simulink model "EMT"  (R2024b)
settings: Solver=ode5  StartTime=0.0  StopTime=1500  FixedStep=0.002  RelTol=1e-3
PreLoadFcn:
  | parameter;
InitFcn:
  | parameter;
StopFcn:
  | save('result.mat');
values from neighbouring files (symbols this model uses):
  A = 7.3    [parameter.m]
  a11 = (1+k1)*(1+k2)/k1/k2/iq    (= 1.54241568346)    [parameter.m]
  a11_L = a11    (= 1.54241568346)    [parameter.m]
  a12 = -(1+k1+k2)*(1+k3)/k1/k2    (= -3.86074191629)    [parameter.m]
  a12_L = a11*(1+k3+k4)/(1+k3)    (= 2.43173643789)    [parameter.m]
  a21 = -(1+k2)/k1/iq    (= -1.04963112005)    [parameter.m]
  a22 = (1+k1+k2)/k1    (= 2.46948356808)    [parameter.m]
  B = 2.71    [parameter.m]
  b11 = 0    [parameter.m]
  b12 = (1+k3)    (= 3.33)    [parameter.m]
  b21 = (1+k2)/iq    (= 2.23571428571)    [parameter.m]
  b22 = -k2    (= -2.13)    [parameter.m]
  C1_shift = 200    [parameter.m]
  Cb = 70    [parameter.m]
  Cd = 0.6    [parameter.m]
  eff_generator = eff_motor    [parameter.m]
  eff_motor = [0.80 0.80 0.84 0.84 0.83 0.85 0.83 0.83 0.83 0.80 0.80 0.80 ... (first row only)    [parameter.m]
  ele_map = [10.00,11.46,14.13,19.24,20.94,23.21,20.29,20.23,22.28,17.66,16.24,18.95,20.79,16.98,18.22,16.52,18.29,20.67,20.82,23.14,23.36,21.30,17.71,20.26,19.53,21.18,23.13,22.79,19.35,16.77,20.50,19.02,20.56,21.90,23.91,20.40,18.45,22.70,22.38,22.48,21.84,17.76,20.13,22.61,19.35,19.36,21.56,20.37,18.38,17.96,18.38,17.24,18.99,22.31,23.50,18.24,22.11,20.73,20.35,18.91,22.88,20.92,18.75,16.85,21.94,17.80,19. ...(+2007 chars)    [parameter.m]
  Fb_max = 5.5*mass    (= 247500)    [parameter.m]
  ic = 4.42    [parameter.m]
  JA = 0.4    [parameter.m]
  JB = JA    (= 0.4)    [parameter.m]
  Jc3r4 = 1e-2    (= 0.01)    [parameter.m]
  Je = 2.5    [parameter.m]
  Jh = 1e-2    (= 0.01)    [parameter.m]
  kh = 2.88    [parameter.m]
  kt = 1.83    [parameter.m]
  L = 4.472    [parameter.m]
  mass = 45000    [parameter.m]
  miu_max = 0.8    [parameter.m]
  n_generator = n_motor    [parameter.m]
  n_motor = [0 0.1 0.25 0.4 0.55 0.7 0.85 1 1.15 1.3 1.45 2.2]*3185    [parameter.m]
  nA_map = [-6000:50:-3250 -3200 0 3200 3250:50:6000]    [parameter.m]    (also in plot_result.m = [-7000:50:-3250 -3200 0 3200 3250:50:7000])
  nA_max = max(nA_map)    [parameter.m]
  nA_min = min(nA_map)    [parameter.m]
  nB_map = nA_map    [parameter.m]    (also in plot_result.m = [-7000:50:-3250 -3200 0 3200 3250:50:7000])
  nB_max = nA_max    [parameter.m]
  nB_min = nA_min    [parameter.m]
  ne_idl = 3000    [parameter.m]
  ne_map = [1600,1700,1800,1900,2000,2100,2200,2300,2400,2500,2600,2700,2800,2900,3000,3100,3200,3300,3400,3500,3600,3700,3800,3900,4000,4100,4200,4500]    [parameter.m]
  ne_max = 4200    [parameter.m]
  ne_min = 1600    [parameter.m]
  ne_start = 200    [parameter.m]
  nZ_map = [-8000:50:-4850 -4800 0 4800 4850:50:8000]    [parameter.m]
  Pb_epr = [-45 -45 -40 -30 0 30 40 45 45]    [parameter.m]
  Pb_max = [0 40 45 45 45]    [parameter.m]
  Pb_min = [-45 -45 -45 -40 0]    [parameter.m]
  Pe_ass = 210+20    (= 230)    [parameter.m]
  Pe_max = 1103    [parameter.m]
  PN0 = 0    [parameter.m]
  R_map = [0.90 0.89 0.90 0.91 0.92 0.93 0.94 0.95 0.96 0.97 0.98]/10    [parameter.m]
  rz = 0.318    [parameter.m]
  SOC0 = 60    [parameter.m]
  SOC_epr = [30 31 50 59 60 61 70 79 80]    [parameter.m]
  SOC_map = 0:10:100    [parameter.m]
  T_generator = T_motor    [parameter.m]
  T_motor = [0 0.3 0.8 1.3 1.8 2.3 2.8]/1.8*1110    [parameter.m]
  TA_max_map = [370*9549./(6000:-50:3250) 1110 1110 1110 370*9549./(3250:50:6000)]    [parameter.m]    (also in plot_result.m = [370*9549./(7000:-50:3250) 1100 1100 1100 370*9549./(3250:50)
  TA_min_map = -TA_max_map    [parameter.m]
  TAf = 0    [parameter.m]
  TB_max_map = TA_max_map    [parameter.m]    (also in plot_result.m = [370*9549./(7000:-50:3250) 1110 1110 1110 370*9549./(3250:50)
  TB_min_map = TA_min_map    [parameter.m]
  TBf = TAf    (= 0)    [parameter.m]
  Te_map = [0,599,798,998,1168,1324,1495,1660,1822,1970,2106,2235,2355,2458,2508,2543,2565,2606,2613,2649,2658,2689,2701,2707,2719,2724,2728,2740,2743,2754]    [parameter.m]
  Te_max_map = [1168,1324,1495,1660,1822,1970,2106,2235,2355,2458,2543,2606,2658,2701,2728,2743,2754,2743,2740,2724,2719,2707,2689,2649,2613,2565,2508,998]    [parameter.m]
  Te_start = 1600    [parameter.m]
  Tef = 100    [parameter.m]
  Time = 0:0.1:200    [parameter.m]
  Time_ele = 0:4:1600    [parameter.m]
  TS_A = 0.2    [parameter.m]
  TS_B = TS_A    (= 0.2)    [parameter.m]
  TS_C0 = 0.2    [parameter.m]
  TS_C1 = 0.2    [parameter.m]
  Ts_e = 0.1    [parameter.m]
  TS_Z1 = 0.2    [parameter.m]
  TS_Z2 = 0.2    [parameter.m]
  TZ_max_map = [450*9549./(8000:-50:4850) 1000 1000 1000 450*9549./(4850:50:8000)]    [parameter.m]
  TZ_min_map = -TZ_max_map    [parameter.m]
  Uoc_map = [3.258,3.668,3.733,3.783,3.833,3.877,3.912,3.941,3.973,4.013,4.200]*250    [parameter.m]
  v_cyc = 0.*(0<=Time&Time<11)+(3.75.*Time-41.25).*(11<=Time&Time<15)+15.*(15<=Time&Time<23)+(-3.*Time+84).*(23<=Time&Time<28)+0.*(28<=Time&Time<49)+(8.*Time/3-392/3).*(49<=Time&Time<61)+32.*(61<=Time&Time<85)+(-32.*Time/11+3072/11).*(85<=Time&Time<96)+0.*(96<=Time&Time<117)+(25.*Time/13-2925/13).*(117<=Time&Time<143)+50.*(143<=Time&Time<155)+(-15.*Time/8+2725/8).*(155<=Time&Time<163)+35.*(163<=Time&Time<17 ...(+70 chars)    [parameter.m]
  V_Shift12 = 32    [parameter.m]
  V_Shift21 = 25    [parameter.m]
  Voltage_epr = [750 760 900 1000 1050]    [parameter.m]
  Y_engine = 0.955    [parameter.m]
  Yc = 0.98    [parameter.m]
  Yh = 0.96    [parameter.m]
  Z1_shift = 200    [parameter.m]
  Z2_shift = 200    [parameter.m]
undefined symbols (not defined in the file or in its folder): sigbuilder_block
libraries: fl_lib x82, nesl_utility x55, simulink x49, sdl_lib x10, simulink_need_slupdate x6, powerlib_extras x1
(part 3 of 6)

== system EMT/Control Unit/Control/Power Distribution/Feasible Control Range ==
  stage : Inport
  ne_act : Inport  Port=2
  v_act : Inport  Port=3
  Memory1 : Memory
  Memory5 : Memory
  State Calculation : Subsystem
  State Predition : Subsystem
  stage_k : Outport
  ne_k : Outport  Port=2
  no_k : Outport  Port=3
  Te_k : Outport  Port=4
  TA_k : Outport  Port=5
  TB_k : Outport  Port=6
  wires:
  State Predition/3(no_k) -> no_k/1
  State Predition/4(Te_k) -> Te_k/1
  State Predition/5(TA_k) -> TA_k/1
  State Predition/6(TB_k) -> TB_k/1
  State Predition/2(ne_k) -> ne_k/1
  State Predition/1(stage_k) -> stage_k/1
  ne_act/1 -> Memory5/1
  stage/1 -> State Calculation/1(s)
  v_act/1 -> Memory1/1
  Memory5/1 -> State Calculation/2(ne)
  Memory1/1 -> State Calculation/3(v_act)
  State Calculation/1(stage) -> State Predition/1(stage)
  State Calculation/2(ne_act) -> State Predition/2(ne_act)
  State Calculation/3(nA_act) -> State Predition/3(nA_act)
  State Calculation/4(nB_act) -> State Predition/4(nB_act)
  State Calculation/5(no_act) -> State Predition/5(no_act)

== system EMT/Control Unit/Control/Power Distribution/Oil Control ==
  Demux : Demux
      settings: DisplayOption=none
  Transfer Fcn1 : TransferFcn  Denominator=[TS_C0 1]
  Transfer Fcn2 : TransferFcn  Denominator=[TS_Z1 1]
  Transfer Fcn3 : TransferFcn  Denominator=[TS_Z2 1]
  Transfer Fcn4 : TransferFcn  Denominator=[TS_C1 1]
  tag scope: Press_C0=global, Press_C1=global, Press_Z1=global, Press_Z2=global
  wires:
  Transfer Fcn1/1 -> [Press_C0]
  Transfer Fcn2/1 -> [Press_Z1]
  Demux/1 -> Transfer Fcn1/1
  Demux/4 -> Transfer Fcn4/1
  Demux/3 -> Transfer Fcn3/1
  Demux/2 -> Transfer Fcn2/1
  Transfer Fcn4/1 -> [Press_C1]
  Transfer Fcn3/1 -> [Press_Z2]
  [Press] -> Demux/1

== system EMT/Control Unit/Control/Power Distribution/Optimal Power Distribution ==
  Pe_com : Inport
  pedal : Inport  Port=2
  stage_k : Inport  Port=3
  ne_k : Inport  Port=4
  no_k : Inport  Port=5
  Te_k : Inport  Port=6
  TA_k : Inport  Port=7
  TB_k : Inport  Port=8
  PN_k : Inport  Port=9
  sd_ne : Inport  Port=10
  Demux : Demux
  "Optimization " : MATLAB Function  TreatAsAtomicUnit=on  SystemSampleTime=0.02
  Rate Transition2 : RateTransition
  Subsystem : Subsystem  mask{Parameter1=on}
      mask prompts: Parameter1 "11"
  ZD_k : Constant
  ne_ref : Outport
  Te_ref : Outport  Port=2
  TA_ref : Outport  Port=3
  TB_ref : Outport  Port=4
  wires:
  Demux/1 -> ne_ref/1
  "Optimization "/1(y) -> Rate Transition2/1
  pedal/1 -> Subsystem/2(In2)
  Pe_com/1 -> Subsystem/1(In1)
  ZD_k/1 -> Subsystem/3(In3)
  ne_k/1 -> Subsystem/5(In5)
  no_k/1 -> Subsystem/6(In6)
  Te_k/1 -> Subsystem/7(In7)
  TA_k/1 -> Subsystem/8(In8)
  TB_k/1 -> Subsystem/9(In9)
  PN_k/1 -> Subsystem/10(In10)
  Demux/4 -> TB_ref/1
  Demux/3 -> TA_ref/1
  Demux/2 -> Te_ref/1
  Subsystem/1(Out) -> "Optimization "/1(u)
  stage_k/1 -> Subsystem/4(In4)
  Rate Transition2/1 -> Demux/1
  sd_ne/1 -> Subsystem/11(In11)

== system EMT/Control Unit/Control/Power Distribution/Pedal Interpretation ==
  Pedal : Inport
  Brake Control : Subsystem
  Data : Subsystem
  Engine Power Requirement : Subsystem
  Subsystem7 : Subsystem
  Subsystem8 : Subsystem
  Fb_ref : Outport
  Pe_com : Outport  Port=2
  wires:
  Engine Power Requirement/1(Pe_com) -> Pe_com/1, Data/3(Pe_com)
  Pedal/1 -> Subsystem7/1(0), Subsystem8/1(0)
  Subsystem7/1(1) -> Engine Power Requirement/1(Acc_pedal), Data/2(Acc_pedal)
  Subsystem8/1(1) -> Brake Control/1(Dec_pedal), Data/1(Dec_pedal)
  Brake Control/1(Fb_ref) -> Fb_ref/1

== system EMT/Control Unit/Control/Power Distribution/Subsystem ==
  Discrete PID Controller : powerlib_extras/Discrete  Control Blocks/Discrete PID Controller  Kp=0.5  Ki=0.1  Kd=0  TcD=1  Par_Limits=[200 -200]  Init=0  Ts=0.5
  Sum : Sum  Inputs=|+-
  sd_ne : Outport
  wires:
  [ne_act] -> Sum/2
  Sum/1 -> Discrete PID Controller/1
  Discrete PID Controller/1 -> sd_ne/1
  [ne_ref] -> Sum/1

== system EMT/Control Unit/Control/Prepare Stage/brack force ==
  Constant1 : Constant  Value=Fb_max
  Fb_com : Outport
  wires:
  Constant1/1 -> Fb_com/1

== system EMT/Control Unit/Control/Prepare Stage/clutches condition ==
  Mux1 : Mux
  Subsystem : Subsystem
  Subsystem1 : Subsystem
  Subsystem2 : Subsystem
  Subsystem3 : Subsystem
  clutch_com : Outport
  wires:
  Subsystem/1(C0) -> Mux1/1
  Subsystem2/1(C1) -> Mux1/4
  Subsystem1/1(Z2) -> Mux1/3
  Subsystem3/1(Z1) -> Mux1/2
  Mux1/1 -> clutch_com/1

== system EMT/Control Unit/Control/Prepare Stage/engine swich ==
  Compare To Constant2 : simulink/Logic and Bit Operations/Compare To Constant  relop=>  const=ne_start  OutDataTypeStr=uint8
  Constant : Constant
  Memory2 : Memory
  Triggered Subsystem : Subsystem  TreatAsAtomicUnit=on
  engine_swich : Outport
  wires:
  Triggered Subsystem/1(Out1) -> engine_swich/1
  Constant/1 -> Triggered Subsystem/1(In1)
  Memory2/1 -> Compare To Constant2/1
  [ne_act] -> Memory2/1
  Compare To Constant2/1 -> Triggered Subsystem/Trigger

== system EMT/Control Unit/Control/Prepare Stage/engine torque ==
  Subsystem1 : Subsystem
  Te_com : Outport
  wires:
  Subsystem1/1(Te_com) -> Te_com/1
  [ne_act] -> Subsystem1/1(ne_act)

== system EMT/Control Unit/Control/Prepare Stage/motorA torque ==
  Constant2 : Constant  Value=0
  Subsystem : Subsystem
  Switch : Switch  Criteria=u2 > Threshold  Threshold=0.1  SaturateOnIntegerOverflow=off  InputSameDT=off
  TA_com1 : Subsystem
  TA_com : Outport
  wires:
  Switch/1 -> TA_com/1
  Subsystem/1(Judge) -> Switch/2
  Constant2/1 -> Switch/3
  TA_com1/1(TA_com) -> Switch/1

== system EMT/Control Unit/Control/Prepare Stage/motorB torque ==
  Lookup Table : Lookup  InputValues=nB_map  Table=TB_max_map*1.5  SaturateOnIntegerOverflow=off
  Lookup Table1 : Lookup  InputValues=nB_map  Table=TB_min_map*1.5  SaturateOnIntegerOverflow=off
  Saturation Dynamic : simulink/Discontinuities/Saturation Dynamic  OutMin=[]  OutMax=[]  OutDataTypeStr=Inherit: Same as second input  OutDataType=sfix(16)  OutScaling=2^-10  DoSatur=off
  Saturation1 : Saturate  UpperLimit=max(nB_map)  LowerLimit=min(nB_map)
  Saturation2 : Saturate  UpperLimit=max(nB_map)  LowerLimit=min(nB_map)
  Subsystem1 : Subsystem
  TB_com : Outport
  wires:
  Saturation Dynamic/1 -> TB_com/1
  [nB_act] -> Subsystem1/1(nB_act), Saturation1/1, Saturation2/1
  Lookup Table/1 -> Saturation Dynamic/1
  Lookup Table1/1 -> Saturation Dynamic/3
  Saturation1/1 -> Lookup Table/1
  Saturation2/1 -> Lookup Table1/1
  Subsystem1/1(TB_com) -> Saturation Dynamic/2

== system EMT/Control Unit/Control/Prepare Stage/motorZ torque ==
  Lookup Table : Lookup  InputValues=nZ_map  Table=TZ_max_map  SaturateOnIntegerOverflow=off
  Lookup Table1 : Lookup  InputValues=nZ_map  Table=TZ_min_map  SaturateOnIntegerOverflow=off
  Saturation Dynamic : simulink/Discontinuities/Saturation Dynamic  OutMin=[]  OutMax=[]  OutDataTypeStr=Inherit: Same as second input  OutDataType=sfix(16)  OutScaling=2^-10  DoSatur=off
  Saturation1 : Saturate  UpperLimit=max(nZ_map)  LowerLimit=min(nZ_map)
  Saturation2 : Saturate  UpperLimit=max(nZ_map)  LowerLimit=min(nZ_map)
  Subsystem1 : Subsystem
  TZ_com : Outport
  wires:
  Saturation Dynamic/1 -> TZ_com/1
  [nZ_act] -> Saturation1/1, Saturation2/1, Subsystem1/1(nZ_act)
  Lookup Table/1 -> Saturation Dynamic/1
  Lookup Table1/1 -> Saturation Dynamic/3
  Saturation1/1 -> Lookup Table/1
  Saturation2/1 -> Lookup Table1/1
  Subsystem1/1(TZ_com) -> Saturation Dynamic/2

== system EMT/Control Unit/Control/Shift Stage/EVT1->EVT2 ==
  Mux : Mux  Inputs=7
  brack force : Subsystem
  clutches condition : Subsystem
  engine swich : Subsystem
  engine torque : Subsystem
  motorA torque : Subsystem
  motorB torque : Subsystem
  motorZ torque : Subsystem
  control : Outport
  wires:
  motorB torque/1(TB_com) -> Mux/5
  motorA torque/1(TA_com) -> Mux/4
  engine torque/1(Te_com) -> Mux/3
  Mux/1 -> control/1
  engine swich/1(engine_swich) -> Mux/2
  clutches condition/1(clutch_com) -> Mux/1
  brack force/1(Fb_com) -> Mux/7
  motorZ torque/1(TZ_com) -> Mux/6

== system EMT/Control Unit/Control/Shift Stage/EVT2->EVT1 ==
  Mux : Mux  Inputs=7
  brack force : Subsystem
  clutches condition : Subsystem
  engine swich : Subsystem
  engine torque : Subsystem
  motorA torque : Subsystem
  motorB torque : Subsystem
  motorZ torque : Subsystem
  control : Outport
  wires:
  motorB torque/1(TB_com) -> Mux/5
  motorA torque/1(TA_com) -> Mux/4
  Mux/1 -> control/1
  engine torque/1(Te_com) -> Mux/3
  engine swich/1(engine_swich) -> Mux/2
  clutches condition/1(clutch_com) -> Mux/1
  brack force/1(Fb_com) -> Mux/7
  motorZ torque/1(TZ_com) -> Mux/6

== system EMT/Control Unit/Control/Shift Stage/Shift Judge ==
  1 : Constant
  Add : Sum
  Compare To Constant1 : simulink/Logic and Bit Operations/Compare To Constant  relop=>  const=1  OutDataTypeStr=uint8
  Data Type Conversion1 : DataTypeConversion  SaturateOnIntegerOverflow=off  RndMeth=Floor
  Fcn : Fcn  Expr=V_Shift21+5*u
  Logical Operator1 : Logic  AllPortsSameDT=off  OutDataTypeStr=boolean
  Memory1 : Memory
  Memory2 : Memory
  Memory5 : Memory
  Relational Operator : RelationalOperator  Operator=<=  OutDataTypeStr=boolean  InputSameDT=off
  shift : Outport
  wires:
  Data Type Conversion1/1 -> Add/2
  Fcn/1 -> Relational Operator/2
  Memory1/1 -> Fcn/1
  [Acc_pedal] -> Memory1/1
  Logical Operator1/1 -> Data Type Conversion1/1
  Compare To Constant1/1 -> Logical Operator1/2
  Relational Operator/1 -> Logical Operator1/1
  [v_act] -> Memory2/1
  Memory2/1 -> Relational Operator/1
  [stage] -> Memory5/1
  Memory5/1 -> Compare To Constant1/1
  1/1 -> Add/1
  Add/1 -> shift/1

== system EMT/Control Unit/Control/Stage Judge/EVT1_H Stage ==
  Compare To Constant1 : simulink/Logic and Bit Operations/Compare To Constant  relop=>  const=0.9  OutDataTypeStr=uint8
  Compare To Constant6 : simulink/Logic and Bit Operations/Compare To Constant  relop=>=  const=0.9  OutDataTypeStr=uint8
  Data Type Conversion : DataTypeConversion  SaturateOnIntegerOverflow=off  RndMeth=Floor
  Logical Operator1 : Logic  AllPortsSameDT=off  OutDataTypeStr=boolean
  Memory1 : Memory
  Memory6 : Memory
  Out1 : Outport
  wires:
  Data Type Conversion/1 -> Out1/1
  Logical Operator1/1 -> Data Type Conversion/1
  Memory1/1 -> Compare To Constant1/1
  [Press_C0] -> Memory1/1
  [Press_Z2] -> Memory6/1
  Memory6/1 -> Compare To Constant6/1
  Compare To Constant1/1 -> Logical Operator1/1
  Compare To Constant6/1 -> Logical Operator1/2

== system EMT/Control Unit/Control/Stage Judge/EVT2 Stage ==
  Add : Sum
  Compare To Constant10 : simulink/Logic and Bit Operations/Compare To Constant  relop=>=  const=2  OutDataTypeStr=uint8
  Compare To Constant11 : simulink/Logic and Bit Operations/Compare To Constant  relop=>  const=0.1  OutDataTypeStr=uint8
  Compare To Constant2 : simulink/Logic and Bit Operations/Compare To Constant  relop=<  const=0.9  OutDataTypeStr=uint8
  Compare To Constant3 : simulink/Logic and Bit Operations/Compare To Constant  relop=<=  const=0.1  OutDataTypeStr=uint8
  Compare To Constant4 : simulink/Logic and Bit Operations/Compare To Constant  relop=>=  const=0.9  OutDataTypeStr=uint8
  Data Type Conversion : DataTypeConversion  SaturateOnIntegerOverflow=off  RndMeth=Floor
  Gain : Gain  Gain=3
  Gain1 : Gain  Gain=2
  Logical Operator : Logic  AllPortsSameDT=off  OutDataTypeStr=boolean
  Logical Operator4 : Logic  Inputs=3  AllPortsSameDT=off  OutDataTypeStr=boolean
  Memory{2..4,10..11} (5 alike) : Memory
  Out1 : Outport
  wires:
  Gain1/1 -> Add/1
  Data Type Conversion/1 -> Out1/1
  Add/1 -> Data Type Conversion/1
  Logical Operator4/1 -> Gain1/1
  Gain/1 -> Add/2
  [Press_Z2] -> Memory3/1
  Memory3/1 -> Compare To Constant3/1
  [Press_C1] -> Memory4/1
  Memory4/1 -> Compare To Constant4/1
  Compare To Constant3/1 -> Logical Operator/1
  Compare To Constant4/1 -> Logical Operator/2
  Logical Operator/1 -> Gain/1
  Compare To Constant2/1 -> Logical Operator4/2
  [Press_Z2] -> Memory2/1
  Memory2/1 -> Compare To Constant2/1
  [stage] -> Memory10/1
  Memory10/1 -> Compare To Constant10/1
  Compare To Constant10/1 -> Logical Operator4/1
  [Press_Z2] -> Memory11/1
  Memory11/1 -> Compare To Constant11/1
  Compare To Constant11/1 -> Logical Operator4/3

== system EMT/Control Unit/Control/Stage Judge/Prepare Stage ==
  Constant2 : Constant  Value=0
  Out1 : Outport
  wires:
  Constant2/1 -> Out1/1

== system EMT/Control Unit/Control/Stage Judge/Shift Stage ==
  Compare To Constant5 : simulink/Logic and Bit Operations/Compare To Constant  relop=>  const=0.1  OutDataTypeStr=uint8
  Compare To Constant9 : simulink/Logic and Bit Operations/Compare To Constant  relop=>  const=0.1  OutDataTypeStr=uint8
  Data Type Conversion : DataTypeConversion  SaturateOnIntegerOverflow=off  RndMeth=Floor
  Logical Operator2 : Logic  AllPortsSameDT=off  OutDataTypeStr=boolean
  Memory5 : Memory
  Memory9 : Memory
  Out1 : Outport
  wires:
  Data Type Conversion/1 -> Out1/1
  Logical Operator2/1 -> Data Type Conversion/1
  Compare To Constant5/1 -> Logical Operator2/2
  [Press_C1] -> Memory5/1
  Memory5/1 -> Compare To Constant5/1
  [Press_Z2] -> Memory9/1
  Memory9/1 -> Compare To Constant9/1
  Compare To Constant9/1 -> Logical Operator2/1

== system EMT/Control Unit/Driver/Electric Power Requirement/Subsystem4 ==
  Subsystem4 : Subsystem
  Subsystem6 : Subsystem
  Out1 : Outport
  Out2 : Outport  Port=2
  Out3 : Outport  Port=3
  Out4 : Outport  Port=4
  Out5 : Outport  Port=5
  Out6 : Outport  Port=6
  Out7 : Outport  Port=7
  Out8 : Outport  Port=8
  wires:
  Subsystem4/4(100) -> Out8/1
  Subsystem4/3(10) -> Out7/1
  Subsystem4/2(0.01) -> Out6/1
  Subsystem4/1(0.1) -> Out5/1
  Subsystem6/4(4) -> Out4/1
  Subsystem6/3(3) -> Out3/1
  Subsystem6/2(2) -> Out2/1
  Subsystem6/1(1) -> Out1/1

== system EMT/Control Unit/Driver/Electric Power Requirement/Subsystem6 ==
  Add : Inport
  Sub : Inport  Port=2
  0.1 : Inport  Port=3
  10 : Inport  Port=4
  0.2 : InportShadow  Port=3
  1 : InportShadow  Port=4
  Add1 : Sum  Inputs=++-
  Memory1 : Memory
  Saturation : Saturate  UpperLimit=800  LowerLimit=0
  Subsystem : Subsystem
  Subsystem1 : Subsystem
  Transfer Fcn2 : TransferFcn  Denominator=[0.05 1]
  Power : Outport
  wires:
  Add1/1 -> Memory1/1, Saturation/1
  Memory1/1 -> Add1/1
  Subsystem1/1(power--) -> Add1/3
  Saturation/1 -> Transfer Fcn2/1
  Subsystem/1(power++) -> Add1/2
  0.1/1 -> Subsystem/1(0.1)
  Add/1 -> Subsystem/2(Add)
  10/1 -> Subsystem/3(10)
  Sub/1 -> Subsystem1/2(Sub)
  1/1 -> Subsystem1/3(10)
  0.2/1 -> Subsystem1/1(0.1)
  Transfer Fcn2/1 -> Power/1

== system EMT/Control Unit/Driver/Gears/Subsystem ==
  Add : Inport
  Sub : Inport  Port=2
  Add1 : Sum  Inputs=++-
  Data Type Conversion : DataTypeConversion  SaturateOnIntegerOverflow=off  RndMeth=Floor
  Data Type Conversion1 : DataTypeConversion  SaturateOnIntegerOverflow=off  RndMeth=Floor
  Memory1 : Memory  InitialCondition=1
  Memory2 : Memory
  Memory3 : Memory
  Relational Operator : RelationalOperator  Operator=~=  OutDataTypeStr=boolean  InputSameDT=off
  Relational Operator1 : RelationalOperator  Operator=~=  OutDataTypeStr=boolean  InputSameDT=off
  Saturation : Saturate  UpperLimit=4  LowerLimit=0
  Gear : Outport
  wires:
  Add1/1 -> Memory1/1, Saturation/1
  Memory1/1 -> Add1/1
  Memory2/1 -> Relational Operator/2
  Add/1 -> Relational Operator/1, Memory2/1
  Memory3/1 -> Relational Operator1/2
  Sub/1 -> Relational Operator1/1, Memory3/1
  Relational Operator1/1 -> Data Type Conversion/1
  Relational Operator/1 -> Data Type Conversion1/1
  Data Type Conversion/1 -> Add1/3
  Data Type Conversion1/1 -> Add1/2
  Saturation/1 -> Gear/1

== system EMT/Control Unit/Driver/Gears/Subsystem1 ==
  11 : Constant
  21 : Constant  Value=2
  22 : Constant  Value=3
  31 : Constant  Value=4
  1 : Outport
  2 : Outport  Port=2
  3 : Outport  Port=3
  4 : Outport  Port=4
  wires:
  11/1 -> 1/1
  21/1 -> 2/1
  22/1 -> 3/1
  31/1 -> 4/1

== system EMT/Control Unit/Driver/Grade Angle/Subsystem4 ==
  Subsystem4 : Subsystem
  Subsystem6 : Subsystem
  Out1 : Outport
  Out2 : Outport  Port=2
  Out3 : Outport  Port=3
  Out4 : Outport  Port=4
  Out5 : Outport  Port=5
  Out6 : Outport  Port=6
  Out7 : Outport  Port=7
  Out8 : Outport  Port=8
  wires:
  Subsystem4/4(100) -> Out8/1
  Subsystem4/3(10) -> Out7/1
  Subsystem4/2(0.01) -> Out6/1
  Subsystem4/1(0.1) -> Out5/1
  Subsystem6/4(4) -> Out4/1
  Subsystem6/3(3) -> Out3/1
  Subsystem6/2(2) -> Out2/1
  Subsystem6/1(1) -> Out1/1

== system EMT/Control Unit/Driver/Grade Angle/Subsystem6 ==
  Add : Inport
  Sub : Inport  Port=2
  0.1 : Inport  Port=3
  10 : Inport  Port=4
  0.2 : InportShadow  Port=3
  1 : InportShadow  Port=4
  Add1 : Sum  Inputs=++-
  Memory1 : Memory
  Saturation : Saturate  UpperLimit=40  LowerLimit=-40
  Subsystem : Subsystem
  Subsystem1 : Subsystem
  Transfer Fcn1 : TransferFcn  Denominator=[0.02 1]
  angle : Outport
  wires:
  Add1/1 -> Memory1/1, Saturation/1
  Memory1/1 -> Add1/1
  Subsystem1/1(angle-) -> Add1/3
  Saturation/1 -> Transfer Fcn1/1
  Subsystem/1(angle++) -> Add1/2
  0.1/1 -> Subsystem/1(0.1)
  Add/1 -> Subsystem/2(Add)
  10/1 -> Subsystem/3(10)
  Sub/1 -> Subsystem1/2(Sub)
  1/1 -> Subsystem1/3(10)
  0.2/1 -> Subsystem1/1(0.1)
  Transfer Fcn1/1 -> angle/1

== system EMT/Control Unit/Driver/Ground Resistance Coefficient/Road ==
  Memory1 : Memory
  Multiport Switch : MultiPortSwitch  DataPortOrder=Zero-based contiguous  Inputs=4  zeroidx=on  SaturateOnIntegerOverflow=off  InputSameDT=off
  Subsystem : Subsystem
  Subsystem1 : Subsystem
  Subsystem2 : Subsystem
  Subsystem3 : Subsystem
  Subsystem4 : Subsystem
  fg : Outport
  wires:
  Memory1/1 -> Subsystem2/1(In1), Subsystem/1(In)
  Subsystem3/1(Out1) -> Multiport Switch/4
  Subsystem2/1(Out1) -> Multiport Switch/3
  Subsystem1/1(Out1) -> Multiport Switch/2
  Subsystem/1(Judge) -> Multiport Switch/1
  Subsystem4/1(Out1) -> Multiport Switch/5
  Multiport Switch/1 -> fg/1
  [Pedal] -> Memory1/1

== system EMT/Control Unit/Driver/Ground Resistance Coefficient/Road1 ==
  1-D Lookup Table : Lookup_n-D  NumberOfTableDimensions=1  BreakpointsForDimension1=[-1 0 0.8 0.9 1]  Table=[10 5 2 1 0.8]  RndMeth=Simplest
  1-D Lookup Table1 : Lookup_n-D  NumberOfTableDimensions=1  BreakpointsForDimension1=[0 10 30 50 60 70 80 90]  Table=[0.16 0.16 0.12 0.10 0.08 0.06 0.05 0.05]  RndMeth=Simplest
  Memory1 : Memory
  Memory2 : Memory
  Product : Product  RndMeth=Zero
  fg : Outport
  wires:
  [Pedal] -> Memory1/1
  [v_act] -> Memory2/1
  Memory2/1 -> 1-D Lookup Table1/1
  Memory1/1 -> 1-D Lookup Table/1
  1-D Lookup Table/1 -> Product/1
  1-D Lookup Table1/1 -> Product/2
  Product/1 -> fg/1

== system EMT/Control Unit/Driver/Ground Resistance Coefficient/Subsystem2 ==
  Subsystem4 : Subsystem
  Subsystem6 : Subsystem
  Out1 : Outport
  Out2 : Outport  Port=2
  Out3 : Outport  Port=3
  Out4 : Outport  Port=4
  Out5 : Outport  Port=5
  Out6 : Outport  Port=6
  Out7 : Outport  Port=7
  Out8 : Outport  Port=8
  wires:
  Subsystem6/1(1) -> Out1/1
  Subsystem6/2(2) -> Out2/1
  Subsystem6/3(3) -> Out3/1
  Subsystem6/4(4) -> Out4/1
  Subsystem4/1(0.1) -> Out5/1
  Subsystem4/2(0.01) -> Out6/1
  Subsystem4/3(10) -> Out7/1
  Subsystem4/4(100) -> Out8/1

== system EMT/Control Unit/Driver/Ground Resistance Coefficient/Subsystem3 ==
  Add : Inport
  Sub : Inport  Port=2
  0.1 : Inport  Port=3
  10 : Inport  Port=4
  0.2 : InportShadow  Port=3
  1 : InportShadow  Port=4
  Add1 : Sum  Inputs=++-
  Memory1 : Memory  InitialCondition=0.04
  Subsystem : Subsystem
  Subsystem1 : Subsystem
  fg : Outport
  wires:
  0.2/1 -> Subsystem1/1(0.1)
  1/1 -> Subsystem1/3(10)
  Sub/1 -> Subsystem1/2(Sub)
  10/1 -> Subsystem/3(10)
  Add/1 -> Subsystem/2(Add)
  0.1/1 -> Subsystem/1(0.1)
  Subsystem/1(fg++) -> Add1/2
  Subsystem1/1(fg--) -> Add1/3
  Memory1/1 -> Add1/1
  Add1/1 -> fg/1, Memory1/1

== system EMT/Control Unit/Driver/Pedal /Auto ==
  1-D Lookup Table1 : Lookup_n-D  NumberOfTableDimensions=1  BreakpointsForDimension1=[-10 -3 -2 -1 0 1 2 10]  Table=[-10 -1 0 0.2 1 2 5 10]  RndMeth=Simplest
  1-D Lookup Table2 : Lookup_n-D  NumberOfTableDimensions=1  BreakpointsForDimension1=[-10 -2 -1 -0.5 0 0.5 1 2 10]  Table=[-1 -0.1 -0.01 -0.001 0 0.001 0.01 0.1 1]  RndMeth=Simplest
  Add : Sum
  Fcn : Fcn  Expr=sqrt(abs((u(2)*mass*9.8*u(1)/3.6/1000/0.8)/Pe_max))
  Memory{1..4} (4 alike) : Memory
  Mux : Mux  Inputs=2
  Product1 : Product  RndMeth=Zero
  Saturation : Saturate  UpperLimit=10  LowerLimit=-10
  Saturation1 : Saturate  UpperLimit=10  LowerLimit=-10
  Pedal : Outport
  wires:
  [v_com] -> Memory1/1
  [fg_act] -> Memory2/1
  Memory1/1 -> Mux/1
  Memory2/1 -> Mux/2
  Mux/1 -> Fcn/1
  Fcn/1 -> Product1/1
  [dv_act] -> Memory3/1
  Memory3/1 -> Saturation/1
  Saturation/1 -> 1-D Lookup Table1/1
  1-D Lookup Table1/1 -> Product1/2
  Product1/1 -> Add/1
  Add/1 -> Pedal/1
  [dv_act] -> Memory4/1
  Memory4/1 -> Saturation1/1
  Saturation1/1 -> 1-D Lookup Table2/1
  1-D Lookup Table2/1 -> Add/2

== system EMT/Control Unit/Driver/Pedal /Signal Builder ==
  Demux : Demux  Tag=STV Demux  Outputs=1
      settings: DisplayOption=none
  FromWs : FromWorkspace  Tag=STV FromWs  VariableName=tuvar
      SigBuilderData=|
      | common.afterFinalStr = 'Extrapolate'
      | common.sampleTime = 0
      | dataSet.timeRange = [0 10]
      | dataSet.name = 'Group 1'
      | sbobj.Groups.Name = 'Group 1'
      | sbobj.Groups.Signals.Name = 'Signal 1'
      | sbobj.Groups.Signals.XData = [0 4 4 6 6 10]
      | sbobj.Groups.Signals.YData = [0.63 0.63 -0.155 -0.155 -1 -1]
  Signal 1 : Outport  Tag=STV Outport
  wires:
  Demux/1 -> Signal 1/1
  FromWs/1 -> Demux/1

== system EMT/Control Unit/Driver/Pedal /Subsystem ==
  1-D Lookup Table : Lookup_n-D  NumberOfTableDimensions=1  BreakpointsForDimension1=Time  Table=v_cyc  RndMeth=Simplest
  Add : Sum  Inputs=+-
  Clock : Clock
  Forward : Constant  Value=85
  Transfer Fcn1 : TransferFcn  Denominator=[1 1]
  dv : Outport
  tag scope: dv_act=global, v_com=global
  wires:
  Add/1 -> [dv_act], dv/1
  Clock/1 -> 1-D Lookup Table/1
  [v_act] -> Add/2
  Transfer Fcn1/1 -> [v_com], Add/1
  1-D Lookup Table/1 -> Transfer Fcn1/1

== system EMT/Control Unit/Driver/Pedal /Subsystem13 ==
  Subsystem4 : Subsystem
  Subsystem6 : Subsystem
  Out1 : Outport
  Out2 : Outport  Port=2
  Out3 : Outport  Port=3
  Out4 : Outport  Port=4
  Out5 : Outport  Port=5
  Out6 : Outport  Port=6
  Out7 : Outport  Port=7
  Out8 : Outport  Port=8
  wires:
  Subsystem4/4(100) -> Out8/1
  Subsystem4/3(10) -> Out7/1
  Subsystem4/2(0.01) -> Out6/1
  Subsystem4/1(0.1) -> Out5/1
  Subsystem6/4(4) -> Out4/1
  Subsystem6/3(3) -> Out3/1
  Subsystem6/2(2) -> Out2/1
  Subsystem6/1(1) -> Out1/1

== system EMT/Control Unit/Driver/Pedal /Subsystem5 ==
  Add : Inport
  Sub : Inport  Port=2
  0.1 : Inport  Port=3
  10 : Inport  Port=4
  0.2 : InportShadow  Port=3
  1 : InportShadow  Port=4
  Add1 : Sum  Inputs=++-
  Memory1 : Memory
  Subsystem : Subsystem
  Subsystem1 : Subsystem
  Pedal : Outport
  wires:
  Add1/1 -> Pedal/1, Memory1/1
  Memory1/1 -> Add1/1
  Subsystem1/1(pedal--) -> Add1/3
  Subsystem/1(pedal++) -> Add1/2
  0.1/1 -> Subsystem/1(0.1)
  Add/1 -> Subsystem/2(Add)
  10/1 -> Subsystem/3(10)
  Sub/1 -> Subsystem1/2(Sub)
  1/1 -> Subsystem1/3(10)
  0.2/1 -> Subsystem1/1(0.1)

== system EMT/Control Unit/Driver/Wheel Angle/Subsystem1 ==
  Subsystem4 : Subsystem
  Subsystem6 : Subsystem
  Out1 : Outport
  Out2 : Outport  Port=2
  Out3 : Outport  Port=3
  Out4 : Outport  Port=4
  Out5 : Outport  Port=5
  Out6 : Outport  Port=6
  Out7 : Outport  Port=7
  Out8 : Outport  Port=8
  wires:
  Subsystem4/4(100) -> Out8/1
  Subsystem4/3(10) -> Out7/1
  Subsystem4/2(0.01) -> Out6/1
  Subsystem4/1(0.1) -> Out5/1
  Subsystem6/4(4) -> Out4/1
  Subsystem6/3(3) -> Out3/1
  Subsystem6/2(2) -> Out2/1
  Subsystem6/1(1) -> Out1/1

== system EMT/Control Unit/Driver/Wheel Angle/Subsystem2 ==
  Add : Inport
  Sub : Inport  Port=2
  0.1 : Inport  Port=3
  10 : Inport  Port=4
  0.2 : InportShadow  Port=3
  1 : InportShadow  Port=4
  Add1 : Sum  Inputs=++-
  Memory1 : Memory
  Saturation : Saturate  UpperLimit=15  LowerLimit=-15
  Subsystem : Subsystem
  Subsystem1 : Subsystem
  Transfer Fcn1 : TransferFcn  Denominator=[0.02 1]
  wheel : Outport
  wires:
  Add1/1 -> Memory1/1, Saturation/1
  Memory1/1 -> Add1/1
  Subsystem1/1(wheel--) -> Add1/3
  Saturation/1 -> Transfer Fcn1/1
  Subsystem/1(wheel++) -> Add1/2
  0.1/1 -> Subsystem/1(0.1)
  Add/1 -> Subsystem/2(Add)
  10/1 -> Subsystem/3(10)
  Sub/1 -> Subsystem1/2(Sub)
  1/1 -> Subsystem1/3(10)
  0.2/1 -> Subsystem1/1(0.1)
  Transfer Fcn1/1 -> wheel/1

== system EMT/Front Gear/C0/C0/Slip Sensor ==
  Abs : Abs  SaturateOnIntegerOverflow=off
  Ideal Rotational Motion Sensor : fl_lib/Mechanical/Mechanical Sensors/Ideal Rotational Motion Sensor  reference=foundation.enum.MeasurementReference.difference  acceleration_port=false  velocity_port=true  position_port=true  wrap_angle=false  offset=0 rad
  PS-Simulink Converter : nesl_utility/PS-Simulink Converter  PhysicalDomain=network_engine_domain  SubClassName=ps_output  LeftPortType=input  RightPortType=output  PseudoPeriodic=off  Frequencies=[]  VectorFormat=1-D array  Unit=1  AffineConversion=off
  Tire Radius2 : Gain  Gain=30/pi
  In : PMIOPort  Side=Left
  Out : PMIOPort  Port=2  Side=Right
  r/min : Outport
  wires:
  PS-Simulink Converter/1 -> Tire Radius2/1
  Tire Radius2/1 -> Abs/1
  Abs/1 -> r/min/1
  connections:
  PS-Simulink Converter/LConn1 -- Ideal Rotational Motion Sensor/RConn2
  Out/RConn1 -- Ideal Rotational Motion Sensor/RConn1
  In/RConn1 -- Ideal Rotational Motion Sensor/LConn1

== system EMT/Front Gear/C0/Power/Speed Sensor ==
  Ideal Rotational Motion Sensor : fl_lib/Mechanical/Mechanical Sensors/Ideal Rotational Motion Sensor  reference=foundation.enum.MeasurementReference.difference  acceleration_port=false  velocity_port=true  position_port=true  wrap_angle=false  offset=0 rad
  PS-Simulink Converter : nesl_utility/PS-Simulink Converter  PhysicalDomain=network_engine_domain  SubClassName=ps_output  LeftPortType=input  RightPortType=output  PseudoPeriodic=off  Frequencies=[]  VectorFormat=1-D array  Unit=rad/s  AffineConversion=off
  Reference : fl_lib/Mechanical/Rotational Elements/Mechanical Rotational Reference
  Tire Radius2 : Gain  Gain=30/pi
  shaft : PMIOPort  Side=Left
  r/min : Outport
  wires:
  PS-Simulink Converter/1 -> Tire Radius2/1
  Tire Radius2/1 -> r/min/1
  connections:
  PS-Simulink Converter/LConn1 -- Ideal Rotational Motion Sensor/RConn2
  Reference/LConn1 -- Ideal Rotational Motion Sensor/RConn1
  shaft/RConn1 -- Ideal Rotational Motion Sensor/LConn1

== system EMT/Front Gear/C0/Power/Torque Sensor ==
  Ideal Torque Sensor : fl_lib/Mechanical/Mechanical Sensors/Ideal Torque Sensor
  PS-Simulink Converter : nesl_utility/PS-Simulink Converter  PhysicalDomain=network_engine_domain  SubClassName=ps_output  LeftPortType=input  RightPortType=output  PseudoPeriodic=off  Frequencies=[]  VectorFormat=1-D array  Unit=1  AffineConversion=off
  In : PMIOPort  Side=Left
  Out : PMIOPort  Port=2  Side=Right
  Nm : Outport
  wires:
  PS-Simulink Converter/1 -> Nm/1
  connections:
  Ideal Torque Sensor/RConn1 -- Out/RConn1
  In/RConn1 -- Ideal Torque Sensor/LConn1
  PS-Simulink Converter/LConn1 -- Ideal Torque Sensor/RConn2

== system EMT/Front Gear/C0/Power1/Speed Sensor ==
  Ideal Rotational Motion Sensor : fl_lib/Mechanical/Mechanical Sensors/Ideal Rotational Motion Sensor  reference=foundation.enum.MeasurementReference.difference  acceleration_port=false  velocity_port=true  position_port=true  wrap_angle=false  offset=0 rad
  PS-Simulink Converter : nesl_utility/PS-Simulink Converter  PhysicalDomain=network_engine_domain  SubClassName=ps_output  LeftPortType=input  RightPortType=output  PseudoPeriodic=off  Frequencies=[]  VectorFormat=1-D array  Unit=rad/s  AffineConversion=off
  Reference : fl_lib/Mechanical/Rotational Elements/Mechanical Rotational Reference
  Tire Radius2 : Gain  Gain=30/pi
  shaft : PMIOPort  Side=Left
  r/min : Outport
  wires:
  Tire Radius2/1 -> r/min/1
  PS-Simulink Converter/1 -> Tire Radius2/1
  connections:
  shaft/RConn1 -- Ideal Rotational Motion Sensor/LConn1
  Reference/LConn1 -- Ideal Rotational Motion Sensor/RConn1
  PS-Simulink Converter/LConn1 -- Ideal Rotational Motion Sensor/RConn2

== system EMT/Front Gear/C0/Power1/Torque Sensor ==
  Ideal Torque Sensor : fl_lib/Mechanical/Mechanical Sensors/Ideal Torque Sensor
  PS-Simulink Converter : nesl_utility/PS-Simulink Converter  PhysicalDomain=network_engine_domain  SubClassName=ps_output  LeftPortType=input  RightPortType=output  PseudoPeriodic=off  Frequencies=[]  VectorFormat=1-D array  Unit=1  AffineConversion=off
  In : PMIOPort  Side=Left
  Out : PMIOPort  Port=2  Side=Right
  Nm : Outport
  wires:
  PS-Simulink Converter/1 -> Nm/1
  connections:
  PS-Simulink Converter/LConn1 -- Ideal Torque Sensor/RConn2
  In/RConn1 -- Ideal Torque Sensor/LConn1
  Ideal Torque Sensor/RConn1 -- Out/RConn1

== system EMT/Power Coupler /C1/C2/Slip Sensor ==
  Abs : Abs  SaturateOnIntegerOverflow=off
  Ideal Rotational Motion Sensor : fl_lib/Mechanical/Mechanical Sensors/Ideal Rotational Motion Sensor  reference=foundation.enum.MeasurementReference.difference  acceleration_port=false  velocity_port=true  position_port=true  wrap_angle=false  offset=0 rad
  PS-Simulink Converter : nesl_utility/PS-Simulink Converter  PhysicalDomain=network_engine_domain  SubClassName=ps_output  LeftPortType=input  RightPortType=output  PseudoPeriodic=off  Frequencies=[]  VectorFormat=1-D array  Unit=1  AffineConversion=off
  Tire Radius2 : Gain  Gain=30/pi
  In : PMIOPort  Side=Left
  Out : PMIOPort  Port=2  Side=Right
  r/min : Outport
  wires:
  Abs/1 -> r/min/1
  Tire Radius2/1 -> Abs/1
  PS-Simulink Converter/1 -> Tire Radius2/1
  connections:
  In/RConn1 -- Ideal Rotational Motion Sensor/LConn1
  Out/RConn1 -- Ideal Rotational Motion Sensor/RConn1
  PS-Simulink Converter/LConn1 -- Ideal Rotational Motion Sensor/RConn2

== system EMT/Power Coupler /C1/Power/Speed Sensor ==
  Ideal Rotational Motion Sensor : fl_lib/Mechanical/Mechanical Sensors/Ideal Rotational Motion Sensor  reference=foundation.enum.MeasurementReference.difference  acceleration_port=false  velocity_port=true  position_port=true  wrap_angle=false  offset=0 rad
  PS-Simulink Converter : nesl_utility/PS-Simulink Converter  PhysicalDomain=network_engine_domain  SubClassName=ps_output  LeftPortType=input  RightPortType=output  PseudoPeriodic=off  Frequencies=[]  VectorFormat=1-D array  Unit=rad/s  AffineConversion=off
  Reference : fl_lib/Mechanical/Rotational Elements/Mechanical Rotational Reference
  Tire Radius2 : Gain  Gain=30/pi
  shaft : PMIOPort  Side=Left
  r/min : Outport
  wires:
  Tire Radius2/1 -> r/min/1
  PS-Simulink Converter/1 -> Tire Radius2/1
  connections:
  shaft/RConn1 -- Ideal Rotational Motion Sensor/LConn1
  Reference/LConn1 -- Ideal Rotational Motion Sensor/RConn1
  PS-Simulink Converter/LConn1 -- Ideal Rotational Motion Sensor/RConn2

== system EMT/Power Coupler /C1/Power/Torque Sensor ==
  Ideal Torque Sensor : fl_lib/Mechanical/Mechanical Sensors/Ideal Torque Sensor
  PS-Simulink Converter : nesl_utility/PS-Simulink Converter  PhysicalDomain=network_engine_domain  SubClassName=ps_output  LeftPortType=input  RightPortType=output  PseudoPeriodic=off  Frequencies=[]  VectorFormat=1-D array  Unit=1  AffineConversion=off
  In : PMIOPort  Side=Left
  Out : PMIOPort  Port=2  Side=Right
  Nm : Outport
  wires:
  PS-Simulink Converter/1 -> Nm/1
  connections:
  PS-Simulink Converter/LConn1 -- Ideal Torque Sensor/RConn2
  In/RConn1 -- Ideal Torque Sensor/LConn1
  Ideal Torque Sensor/RConn1 -- Out/RConn1

== system EMT/Power Coupler /C1/Power1/Speed Sensor ==
  Ideal Rotational Motion Sensor : fl_lib/Mechanical/Mechanical Sensors/Ideal Rotational Motion Sensor  reference=foundation.enum.MeasurementReference.difference  acceleration_port=false  velocity_port=true  position_port=true  wrap_angle=false  offset=0 rad
  PS-Simulink Converter : nesl_utility/PS-Simulink Converter  PhysicalDomain=network_engine_domain  SubClassName=ps_output  LeftPortType=input  RightPortType=output  PseudoPeriodic=off  Frequencies=[]  VectorFormat=1-D array  Unit=rad/s  AffineConversion=off
  Reference : fl_lib/Mechanical/Rotational Elements/Mechanical Rotational Reference
  Tire Radius2 : Gain  Gain=30/pi
  shaft : PMIOPort  Side=Left
  r/min : Outport
  wires:
  PS-Simulink Converter/1 -> Tire Radius2/1
  Tire Radius2/1 -> r/min/1
  connections:
  PS-Simulink Converter/LConn1 -- Ideal Rotational Motion Sensor/RConn2
  Reference/LConn1 -- Ideal Rotational Motion Sensor/RConn1
  shaft/RConn1 -- Ideal Rotational Motion Sensor/LConn1

== system EMT/Power Coupler /C1/Power1/Torque Sensor ==
  Ideal Torque Sensor : fl_lib/Mechanical/Mechanical Sensors/Ideal Torque Sensor
  PS-Simulink Converter : nesl_utility/PS-Simulink Converter  PhysicalDomain=network_engine_domain  SubClassName=ps_output  LeftPortType=input  RightPortType=output  PseudoPeriodic=off  Frequencies=[]  VectorFormat=1-D array  Unit=1  AffineConversion=off
  In : PMIOPort  Side=Left
  Out : PMIOPort  Port=2  Side=Right
  Nm : Outport
  wires:
  PS-Simulink Converter/1 -> Nm/1
  connections:
  Ideal Torque Sensor/RConn1 -- Out/RConn1
  In/RConn1 -- Ideal Torque Sensor/LConn1
  PS-Simulink Converter/LConn1 -- Ideal Torque Sensor/RConn2

== system EMT/Power Coupler /Z1/Z/Power ==
  Gain1 : Gain  Gain=1/9549
  Product3 : Product  RndMeth=Zero
  Speed Sensor : Subsystem  mask(Speed Sensor){}
      mask help: The speed unit is r/min.
  Torque Sensor : Subsystem  mask(Torque Sensor){}
      mask help: The torque unit is Nm.
  In : PMIOPort  Side=Left
  Out : PMIOPort  Port=2  Side=Right
  kW : Outport
  wires:
  Product3/1 -> kW/1
  Gain1/1 -> Product3/1
  Torque Sensor/1(Nm) -> Gain1/1
  Speed Sensor/1(r/min) -> Product3/2
  connections:
  In/RConn1 -- Torque Sensor/LConn1
  Torque Sensor/RConn1 -- Out/RConn1 -- Speed Sensor/LConn1

== system EMT/Power Coupler /Z1/Z/Power1 ==
  Gain1 : Gain  Gain=1/9549
  Product3 : Product  RndMeth=Zero
  Speed Sensor : Subsystem  mask(Speed Sensor){}
      mask help: The speed unit is r/min.
  Torque Sensor : Subsystem  mask(Torque Sensor){}
      mask help: The torque unit is Nm.
  In : PMIOPort  Side=Left
  Out : PMIOPort  Port=2  Side=Right
  kW : Outport
  wires:
  Speed Sensor/1(r/min) -> Product3/2
  Torque Sensor/1(Nm) -> Gain1/1
  Gain1/1 -> Product3/1
  Product3/1 -> kW/1
  connections:
  Speed Sensor/LConn1 -- Out/RConn1 -- Torque Sensor/RConn1
  In/RConn1 -- Torque Sensor/LConn1

== system EMT/Power Coupler /Z1/Z/Z1 ==
  Press : Inport
  Simulink-PS Converter : nesl_utility/Simulink-PS Converter  PhysicalDomain=network_engine_domain  SubClassName=ps_input  LeftPortType=input  RightPortType=output  PseudoPeriodic=off  Frequencies=[]  NoiseDistribution=none  NoiseParameters=[]  Unit=Pa  AffineConversion=off  FilteringAndDerivatives=filter  SimscapeFilterOrder=1  InputFilterTimeConstant=.001  UdotUserProvided=1
  Slip Sensor : Subsystem  mask(Slip Sensor){}
      mask help: The speed unit is r/min.
  Tire Radius2 : Gain  Gain=2500000
  Z1 : sdl_lib/Clutches/Disc Friction Clutch  geometry_model=2  r_eff=130 mm  d_o=207*2 mm  d_i=174.25*2 mm  nS=12  piston_area=0.0528 m^2  unidirectional=0  friction_model=1  mu_w_vector=[ 0 0.1 0.2 0.3 0.4 0.5 1 2 5 10 100 1000 ] rad/s  temperature_TLU=[280.0, 300.0, 320.0] K  mu_static=0.10  mu_static_vector=[0.4, 0.38, 0.36]  mu_coulomb=0.06  mu_coulomb_vector=[ 0.29 0.28 0.26 0.22 0.21 0.2 0.2 0.19 0.19 0.19 0.19 0.19 ]  mu_coulomb_temp_vector=[0.3, 0.28, 0.25]  mu_coulomb_matrix=[0.34, 0.32, 0.3; 0.3, 0.28, 0.25; 0.25, 0.2, 0.15]  mu_interp_method=1  mu_extrap_method=1  d_f=0.6  w_tol=0.001 rad/s  pressure_min=1930 Pa  mu_visc=0.1580 N*m/(rad/s)  initial_state_locked=0  thermal_mass=25 kJ/K  T_init=300 K
      settings: InternalSimscapePortConfiguration="{\"Bottom\":[],\"Left\":[{\"id\":\"P\",\"label\":\"P\",\"type\":\"input\"},{\"id\":\"B\",\"label\":\"B\",\"type\":\"foundation.mechanical.rotational.rotational\"}],\"Right\":[{\"id\":\"F\",\"label\":\"F\",\"type\":\"foundation.mechanical.rotational.rotational\"}],\"Top\":[]}"
  In : PMIOPort  Side=Left
  Out : PMIOPort  Port=2  Side=Right
  r/min : Outport
  wires:
  Slip Sensor/1(r/min) -> r/min/1
  Press/1 -> Tire Radius2/1
  Tire Radius2/1 -> Simulink-PS Converter/1
  connections:
  Slip Sensor/RConn1 -- Out/RConn1 -- Z1/RConn1
  Slip Sensor/LConn1 -- Z1/LConn2 -- In/RConn1
  Simulink-PS Converter/RConn1 -- Z1/LConn1

== system EMT/Power Coupler /Z2/Z/Power ==
  Gain1 : Gain  Gain=1/9549
  Product3 : Product  RndMeth=Zero
  Speed Sensor : Subsystem  mask(Speed Sensor){}
      mask help: The speed unit is r/min.
  Torque Sensor : Subsystem  mask(Torque Sensor){}
      mask help: The torque unit is Nm.
  In : PMIOPort  Side=Left
  Out : PMIOPort  Port=2  Side=Right
  kW : Outport
  wires:
  Product3/1 -> kW/1
  Gain1/1 -> Product3/1
  Torque Sensor/1(Nm) -> Gain1/1
  Speed Sensor/1(r/min) -> Product3/2
  connections:
  In/RConn1 -- Torque Sensor/LConn1
  Torque Sensor/RConn1 -- Out/RConn1 -- Speed Sensor/LConn1

== system EMT/Power Coupler /Z2/Z/Power1 ==
  Gain1 : Gain  Gain=1/9549
  Product3 : Product  RndMeth=Zero
  Speed Sensor : Subsystem  mask(Speed Sensor){}
      mask help: The speed unit is r/min.
  Torque Sensor : Subsystem  mask(Torque Sensor){}
      mask help: The torque unit is Nm.
  In : PMIOPort  Side=Left
  Out : PMIOPort  Port=2  Side=Right
  kW : Outport
  wires:
  Speed Sensor/1(r/min) -> Product3/2
  Torque Sensor/1(Nm) -> Gain1/1
  Gain1/1 -> Product3/1
  Product3/1 -> kW/1
  connections:
  Speed Sensor/LConn1 -- Out/RConn1 -- Torque Sensor/RConn1
  In/RConn1 -- Torque Sensor/LConn1

== system EMT/Power Coupler /Z2/Z/Z2 ==
  Press : Inport
  Simulink-PS Converter : nesl_utility/Simulink-PS Converter  PhysicalDomain=network_engine_domain  SubClassName=ps_input  LeftPortType=input  RightPortType=output  PseudoPeriodic=off  Frequencies=[]  NoiseDistribution=none  NoiseParameters=[]  Unit=Pa  AffineConversion=off  FilteringAndDerivatives=filter  SimscapeFilterOrder=1  InputFilterTimeConstant=.001  UdotUserProvided=1
  Slip Sensor : Subsystem  mask(Slip Sensor){}
      mask help: The speed unit is r/min.
  Tire Radius2 : Gain  Gain=2500000
  Z2 : sdl_lib/Clutches/Disc Friction Clutch  geometry_model=2  r_eff=130 mm  d_o=189*2 mm  d_i=165.25*2 mm  nS=10  piston_area=0.0264 m^2  unidirectional=0  friction_model=1  mu_w_vector=[ 0 0.1 0.2 0.3 0.4 0.5 1 2 5 10 100 1000 ] rad/s  temperature_TLU=[280.0, 300.0, 320.0] K  mu_static=0.10  mu_static_vector=[0.4, 0.38, 0.36]  mu_coulomb=0.06  mu_coulomb_vector=[ 0.29 0.28 0.26 0.22 0.21 0.2 0.2 0.19 0.19 0.19 0.19 0.19 ]  mu_coulomb_temp_vector=[0.3, 0.28, 0.25]  mu_coulomb_matrix=[0.34, 0.32, 0.3; 0.3, 0.28, 0.25; 0.25, 0.2, 0.15]  mu_interp_method=1  mu_extrap_method=1  d_f=0.6  w_tol=0.001 rad/s  pressure_min=1830 Pa  mu_visc=0.0764 N*m/(rad/s)  initial_state_locked=0  thermal_mass=25 kJ/K  T_init=300 K
      settings: InternalSimscapePortConfiguration="{\"Bottom\":[],\"Left\":[{\"id\":\"P\",\"label\":\"P\",\"type\":\"input\"},{\"id\":\"B\",\"label\":\"B\",\"type\":\"foundation.mechanical.rotational.rotational\"}],\"Right\":[{\"id\":\"F\",\"label\":\"F\",\"type\":\"foundation.mechanical.rotational.rotational\"}],\"Top\":[]}"
  In : PMIOPort  Side=Left
  Out : PMIOPort  Port=2  Side=Right
  r/min : Outport
  wires:
  Slip Sensor/1(r/min) -> r/min/1
  Press/1 -> Tire Radius2/1
  Tire Radius2/1 -> Simulink-PS Converter/1
  connections:
  Slip Sensor/RConn1 -- Out/RConn1 -- Z2/RConn1
  Slip Sensor/LConn1 -- Z2/LConn2 -- In/RConn1
  Simulink-PS Converter/RConn1 -- Z2/LConn1

== system EMT/Vehicle dynamics/vehicle dynamic/vehicle dynamic/Grade Resistance ==
  angle : Inport
  Ground Resistance : Fcn  Expr=0.5*mass*9.8*sin(u)
  Fg : Outport
  wires:
  Ground Resistance/1 -> Fg/1
  angle/1 -> Ground Resistance/1

== system EMT/Vehicle dynamics/vehicle dynamic/vehicle dynamic/Ground Resistance ==
  fg : Inport
  angle : Inport  Port=2
  Ground Resistance : Fcn  Expr=0.5*u(1)*mass*9.8*cos(u(2))
  Mux : Mux  Inputs=2
  Ff : Outport
  wires:
  Ground Resistance/1 -> Ff/1
  Mux/1 -> Ground Resistance/1
  fg/1 -> Mux/1
  angle/1 -> Mux/2

== system EMT/Vehicle dynamics/vehicle dynamic/vehicle dynamic/Mode Judge ==
  v : Inport
  Add : Sum  Inputs=+++
  Compare To Constant1 : simulink/Logic and Bit Operations/Compare To Constant  relop=<  const=-0.1  OutDataTypeStr=uint8
  Compare To Constant2 : simulink/Logic and Bit Operations/Compare To Constant  relop=>  const=0.1  OutDataTypeStr=uint8
  Compare To Constant3 : simulink/Logic and Bit Operations/Compare To Constant  relop=>=  const=-0.1  OutDataTypeStr=uint8
  Compare To Constant4 : simulink/Logic and Bit Operations/Compare To Constant  relop=<=  const=0.1  OutDataTypeStr=uint8
  Data Type Conversion : DataTypeConversion  SaturateOnIntegerOverflow=off  RndMeth=Floor
  Gain : Gain  Gain=3
  Gain1 : Gain  Gain=2
  Gain2 : Gain
  Logical Operator : Logic  AllPortsSameDT=off  OutDataTypeStr=boolean
  F : Outport
  wires:
  Gain1/1 -> Add/2
  Add/1 -> Data Type Conversion/1
  v/1 -> Compare To Constant4/1, Compare To Constant3/1, Compare To Constant2/1, Compare To Constant1/1
  Compare To Constant1/1 -> Gain2/1
  Compare To Constant3/1 -> Logical Operator/1
  Compare To Constant4/1 -> Logical Operator/2
  Compare To Constant2/1 -> Gain1/1
  Logical Operator/1 -> Gain/1
  Data Type Conversion/1 -> F/1
  Gain/1 -> Add/3
  Gain2/1 -> Add/1

== system EMT/Vehicle dynamics/vehicle dynamic/vehicle dynamic/Speed Sensor ==
  Ideal Rotational Motion Sensor : fl_lib/Mechanical/Mechanical Sensors/Ideal Rotational Motion Sensor  reference=foundation.enum.MeasurementReference.difference  acceleration_port=false  velocity_port=true  position_port=true  wrap_angle=false  offset=0 rad
  PS-Simulink Converter : nesl_utility/PS-Simulink Converter  PhysicalDomain=network_engine_domain  SubClassName=ps_output  LeftPortType=input  RightPortType=output  PseudoPeriodic=off  Frequencies=[]  VectorFormat=1-D array  Unit=1  AffineConversion=off
  Reference : fl_lib/Mechanical/Rotational Elements/Mechanical Rotational Reference
  Tire Radius2 : Gain  Gain=30/pi
  shaft : PMIOPort  Side=Left
  r/min : Outport
  wires:
  Tire Radius2/1 -> r/min/1
  PS-Simulink Converter/1 -> Tire Radius2/1
  connections:
  shaft/RConn1 -- Ideal Rotational Motion Sensor/LConn1
  Reference/LConn1 -- Ideal Rotational Motion Sensor/RConn1
  PS-Simulink Converter/LConn1 -- Ideal Rotational Motion Sensor/RConn2

== system EMT/Vehicle dynamics/vehicle dynamic/vehicle dynamic/Steering Resistance ==
  Abs : Abs  SaturateOnIntegerOverflow=off
  Compare To Constant : simulink/Logic and Bit Operations/Compare To Constant  relop=>=  const=10^3  OutDataTypeStr=uint8  ZeroCross=off
  Constant1 : Constant  Value=0
  Memory1 : Memory
  Memory3 : Memory
  Mux : Mux  Inputs=2
  Product2 : Product  RndMeth=Zero
  Sign1 : Signum
  Steering Resistance : Fcn  Expr=miu_max/(0.925+0.15*(u))*mass*9.8*L/4/B
  Switch : Switch  Threshold=0.5  SaturateOnIntegerOverflow=off  InputSameDT=off
  rou : Fcn  Expr=(u(1)+u(2))/(u(1)-u(2)+0.1^10)/2
  Fs : Outport
  wires:
  Steering Resistance/1 -> Product2/1
  Memory3/1 -> Mux/1
  Memory1/1 -> Mux/2
  Mux/1 -> rou/1
  rou/1 -> Abs/1, Compare To Constant/1, Sign1/1
  Abs/1 -> Steering Resistance/1  "rou"
  Compare To Constant/1 -> Switch/2
  Constant1/1 -> Switch/1
  Switch/1 -> Product2/2
  Sign1/1 -> Switch/3
  Product2/1 -> Fs/1
  [v_Left] -> Memory3/1
  [v_Right] -> Memory1/1
